simulink model "grid_forming_dq"  (R2026b)
settings: Solver=ode23tb  StopTime=param.sim.simlength  FixedStep=tc  MaxStep=param.glb_time.tc
values from neighbouring files (symbols this model uses):
  param = struct()    [init_model.m]
undefined symbols (not defined in the file or in its folder): magnitude
libraries: fl_lib x163, nesl_utility x93, igbt_simple_2th_lib x6, single_phase_transformer_lib x3, threephase_inductor_lib x2, dclink_for_two_levels x1, three_phase_pwm_modulator x1, lithium_ion_battery x1, three_phase_rl_load x1
(part 3 of 6)

== system grid_forming_dq/afe_dq_mod1/AFE_control/afe_control/current_ctrl/current_transformation ==
  is_a_pu : Inport
  is_b_pu : Inport  Port=2
  is_c_pu : Inport  Port=3
  alphabeta2xieta : MATLAB Function  TreatAsAtomicUnit=on
  uvw2alphabeta : MATLAB Function  TreatAsAtomicUnit=on
  tag scope: id_eta_pu=scoped, id_xi_pu=scoped
  wires:
  is_c_pu/1 -> uvw2alphabeta/3(w)
  alphabeta2xieta/2(eta) -> [id_eta_pu]  "ieta_pu"
  alphabeta2xieta/1(xi) -> [id_xi_pu]  "ixi_pu"
  is_b_pu/1 -> uvw2alphabeta/2(v)
  uvw2alphabeta/2(beta) -> alphabeta2xieta/2(beta)  "ibeta_pu"
  uvw2alphabeta/1(alpha) -> alphabeta2xieta/1(alpha)  "ialpha_pu"
  [phase_grid_pll] -> alphabeta2xieta/3(gamma)
  is_a_pu/1 -> uvw2alphabeta/1(u)

== system grid_forming_dq/afe_dq_mod1/AFE_control/afe_control/current_ctrl/dq_vector_pi ==
  id : Inport
  id_ref : Inport  Port=2
  iq : Inport  Port=3
  iq_ref : Inport  Port=4
  Sum1 : Sum  Inputs=|-+
  Sum2 : Sum  Inputs=|-+
  bounder1 : Subsystem
  bounder2 : Subsystem
  id/id_ref : Scope  NumInputPorts=2
      settings: ActiveDisplayYMinimum=-0.59440941888164511  ActiveDisplayYMaximum=1.5837925471243963  DataLoggingVariableName=ScopeData4
  iq/iq_ref : Scope  NumInputPorts=2
      settings: ActiveDisplayYMinimum=-1.3392283585411369  ActiveDisplayYMaximum=1.0516657066165265  DataLoggingVariableName=ScopeData5
  pi_d : Subsystem
  pi_q : Subsystem
  switch : Subsystem
  vector lenght : Subsystem
  md_sat : Outport
  mq_sat : Outport  Port=2
  wires:
  bounder2/2(clip) -> switch/2(clip 2)
  vector lenght/2(m) -> bounder1/3(m), bounder2/1(m)
  Sum2/1 -> pi_q/1(iq_tilde)
  pi_d/1(ud_ctrl_out) -> vector lenght/1(md), bounder1/1(md)
  pi_q/1(uq_ctrl_out) -> bounder2/3(mq), vector lenght/2(mq)
  vector lenght/1(m_1) -> bounder1/2(m_1), bounder2/2(m_1)
  switch/1(clip) -> pi_d/2(clip), pi_q/2(clip)
  iq/1 -> Sum2/1, iq/iq_ref/1  "iq"
  Sum1/1 -> pi_d/1(id_tilde)
  bounder1/2(clip) -> switch/1(clip 1)
  bounder1/1(md_sat) -> md_sat/1
  bounder2/1(mq_sat) -> mq_sat/1
  id_ref/1 -> id/id_ref/2, Sum1/2  "id_ref"
  iq_ref/1 -> iq/iq_ref/2, Sum2/2  "iq_ref"
  id/1 -> id/id_ref/1, Sum1/1  "id"

== system grid_forming_dq/afe_dq_mod1/AFE_control/afe_control/current_ctrl/zero_current_ctrl ==
  ualpha_ctrl_afe : Inport
  ubeta_ctrl_afe : Inport  Port=2
  Bus Creator1 : BusCreator  Inputs=3
  Constant : Constant  Value=0
  uabg_ctrl_out : Outport
  wires:
  Bus Creator1/1 -> uabg_ctrl_out/1
  ualpha_ctrl_afe/1 -> Bus Creator1/1  "ualpha_ctrl_afe"
  ubeta_ctrl_afe/1 -> Bus Creator1/2  "ubeta_ctrl_afe"
  Constant/1 -> Bus Creator1/3  "ugamma_ctrl_afe"

== system grid_forming_dq/afe_dq_mod1/AFE_control/afe_control/data_to_worspace_module_1/dq_pll ==
  Bus Creator1 : BusCreator  Inputs=8
  dqPLLs : Outport
  wires:
  [phase_grid_fht_simulink_pll] -> Bus Creator1/5  "phase_grid_fht_simulink_pll"
  [omega_grid_fht_simulink_pll] -> Bus Creator1/6  "omega_grid_fht_simulink_pll"
  [omega_grid_fhtsr_dqpll] -> Bus Creator1/8  "omega_grid_fhtsr_dqpll"
  [phase_grid_fhtsr_dqpll] -> Bus Creator1/7  "phase_grid_fhtsr_dqpll"
  [omega_grid_dqpll_ccaller] -> Bus Creator1/4  "omega_grid_dqpll_ccaller"
  [phase_grid_dqpll_ccaller] -> Bus Creator1/3  "phase_grid_dqpll_ccaller"
  [omega_grid_pu_dqpll] -> Bus Creator1/2  "omega_grid_pu_dqpll"
  [phase_grid_dqpll] -> Bus Creator1/1  "phase_grid_dqpll"
  Bus Creator1/1 -> dqPLLs/1

== system grid_forming_dq/afe_dq_mod1/AFE_control/afe_control/data_to_worspace_module_1/pwr_meter ==
  Bus Creator1 : BusCreator  Inputs=4
  m_pwr_meter : Outport
  wires:
  [u_grid_pu_rms] -> Bus Creator1/2  "u_grid_pu_rms"
  Bus Creator1/1 -> m_pwr_meter/1
  [pwr_act_grid] -> Bus Creator1/3  "pwr_act_grid"
  [pwr_react_grid] -> Bus Creator1/4  "pwr_react_grid"
  [i_grid_pu_rms] -> Bus Creator1/1  "i_grid_pu_rms"

== system grid_forming_dq/afe_dq_mod1/AFE_control/afe_control/dq_neg_vector_pi/bounder1 ==
  md : Inport
  m_1 : Inport  Port=2
  m : Inport  Port=3
  Constant : Constant
  Constant1 : Constant  Value=0
  Divide : Product
  Gain : Gain  Gain=param.afe.ctrl.ixi_pos_ref_lim
  Switch : Switch  Threshold=param.afe.ctrl.ixi_pos_ref_lim  SaturateOnIntegerOverflow=off  InputSameDT=off
  Switch1 : Switch  Threshold=param.afe.ctrl.ixi_pos_ref_lim  SaturateOnIntegerOverflow=off  InputSameDT=off
  md_sat : Outport  VectorParamsAs1DForOutWhenUnconnected=off
  clip : Outport  Port=2  VectorParamsAs1DForOutWhenUnconnected=off
  wires:
  Gain/1 -> Switch1/1
  Switch1/1 -> md_sat/1
  Constant1/1 -> Switch/3
  Constant/1 -> Switch/1
  m/1 -> Switch1/2, Switch/2
  Switch/1 -> clip/1
  Divide/1 -> Gain/1
  m_1/1 -> Divide/1
  md/1 -> Divide/2, Switch1/3

== system grid_forming_dq/afe_dq_mod1/AFE_control/afe_control/dq_neg_vector_pi/bounder2 ==
  m : Inport
  m_1 : Inport  Port=2
  mq : Inport  Port=3
  Constant : Constant
  Constant1 : Constant  Value=0
  Divide : Product
  Gain : Gain  Gain=param.afe.ctrl.ixi_pos_ref_lim
  Switch : Switch  Threshold=param.afe.ctrl.ixi_pos_ref_lim  SaturateOnIntegerOverflow=off  InputSameDT=off
  Switch1 : Switch  Threshold=param.afe.ctrl.ixi_pos_ref_lim  SaturateOnIntegerOverflow=off  InputSameDT=off
  mq_sat : Outport  VectorParamsAs1DForOutWhenUnconnected=off
  clip : Outport  Port=2  VectorParamsAs1DForOutWhenUnconnected=off
  wires:
  Gain/1 -> Switch1/1
  mq/1 -> Switch1/3, Divide/2
  m_1/1 -> Divide/1
  Divide/1 -> Gain/1
  Switch1/1 -> mq_sat/1
  Switch/1 -> clip/1
  m/1 -> Switch/2, Switch1/2
  Constant/1 -> Switch/1
  Constant1/1 -> Switch/3

== system grid_forming_dq/afe_dq_mod1/AFE_control/afe_control/dq_neg_vector_pi/pi_d ==
  id_tilde : Inport
  clip : Inport  Port=2
  1/Ti : Gain  Gain=param.afe.ctrl.kp_ug_ctrl  SaturateOnIntegerOverflow=on  OutDataTypeStr=Inherit: Same as input  ParamDataTypeStr=Inherit: Same as input
  Constant : Constant  Value=0
  Sum2 : Sum  Inputs=+-  SaturateOnIntegerOverflow=on
  Sum4 : Sum  SaturateOnIntegerOverflow=on
  Sum5 : Sum  SaturateOnIntegerOverflow=on
  Switch1 : Switch  Threshold=0.5  SaturateOnIntegerOverflow=off  InputSameDT=off
  Switch2 : Switch  Threshold=0.5  SaturateOnIntegerOverflow=off  InputSameDT=off
  Unit Delay1 : UnitDelay  SampleTime=-1
  Unit Delay2 : UnitDelay  SampleTime=-1
  kp1 : Gain  Gain=param.ctrl.CTRPIFF_CLIP_RELEASE*param.glb_time.ts_inv  SaturateOnIntegerOverflow=on  OutDataTypeStr=Inherit: Same as input  ParamDataTypeStr=Inherit: Same as input
  kp2 : Gain  Gain=param.afe.ctrl.ki_ug_ctrl*param.glb_time.ts_inv  SaturateOnIntegerOverflow=on  OutDataTypeStr=Inherit: Same as input  ParamDataTypeStr=Inherit: Same as input
  ud_out : Outport  VectorParamsAs1DForOutWhenUnconnected=off
  wires:
  Unit Delay1/1 -> [clip]
  Constant/1 -> Switch2/1
  [clip] -> Switch1/2
  [clip] -> Switch2/2
  clip/1 -> Unit Delay1/1
  kp2/1 -> Switch2/3
  Switch2/1 -> Sum4/1
  1/Ti/1 -> Sum5/1
  Unit Delay2/1 -> Sum2/1, kp1/1, Sum4/2
  Sum2/1 -> Switch1/1
  kp1/1 -> Sum2/2
  Sum4/1 -> Switch1/3, Sum5/2
  Switch1/1 -> Unit Delay2/1
  Sum5/1 -> ud_out/1
  id_tilde/1 -> 1/Ti/1, kp2/1

== system grid_forming_dq/afe_dq_mod1/AFE_control/afe_control/dq_neg_vector_pi/pi_q ==
  iq_tilde : Inport
  clip : Inport  Port=2
  1/Ti : Gain  Gain=param.afe.ctrl.kp_ug_ctrl  SaturateOnIntegerOverflow=on  OutDataTypeStr=Inherit: Same as input  ParamDataTypeStr=Inherit: Same as input
  Constant : Constant  Value=0
  Sum2 : Sum  Inputs=+-  SaturateOnIntegerOverflow=on
  Sum4 : Sum  SaturateOnIntegerOverflow=on
  Sum5 : Sum  SaturateOnIntegerOverflow=on
  Switch1 : Switch  Threshold=0.5  SaturateOnIntegerOverflow=off  InputSameDT=off
  Switch2 : Switch  Threshold=0.5  SaturateOnIntegerOverflow=off  InputSameDT=off
  Unit Delay1 : UnitDelay  SampleTime=-1
  Unit Delay2 : UnitDelay  SampleTime=-1
  kp1 : Gain  Gain=param.ctrl.CTRPIFF_CLIP_RELEASE*param.glb_time.ts_inv  SaturateOnIntegerOverflow=on  OutDataTypeStr=Inherit: Same as input  ParamDataTypeStr=Inherit: Same as input
  kp2 : Gain  Gain=param.afe.ctrl.ki_ug_ctrl*param.glb_time.ts_inv  SaturateOnIntegerOverflow=on  OutDataTypeStr=Inherit: Same as input  ParamDataTypeStr=Inherit: Same as input
  Vqs_out : Outport  VectorParamsAs1DForOutWhenUnconnected=off
  wires:
  Sum5/1 -> Vqs_out/1
  Unit Delay1/1 -> [clip]
  iq_tilde/1 -> kp2/1, 1/Ti/1
  Switch1/1 -> Unit Delay2/1
  Sum4/1 -> Switch1/3, Sum5/2
  kp1/1 -> Sum2/2
  Sum2/1 -> Switch1/1
  Unit Delay2/1 -> Sum4/2, kp1/1, Sum2/1
  1/Ti/1 -> Sum5/1
  Switch2/1 -> Sum4/1
  kp2/1 -> Switch2/3
  clip/1 -> Unit Delay1/1
  [clip] -> Switch2/2
  [clip] -> Switch1/2
  Constant/1 -> Switch2/1

== system grid_forming_dq/afe_dq_mod1/AFE_control/afe_control/dq_neg_vector_pi/switch ==
  clip 1 : Inport
  clip 2 : Inport  Port=2
  Constant4 : Constant
  Constant5 : Constant  Value=0
  Sum1 : Sum  SaturateOnIntegerOverflow=on
  Switch : Switch  Threshold=0.5  SaturateOnIntegerOverflow=off  InputSameDT=off
  clip : Outport  VectorParamsAs1DForOutWhenUnconnected=off
  wires:
  clip 2/1 -> Sum1/2
  clip 1/1 -> Sum1/1
  Sum1/1 -> Switch/2
  Constant4/1 -> Switch/1
  Switch/1 -> clip/1
  Constant5/1 -> Switch/3

== system grid_forming_dq/afe_dq_mod1/AFE_control/afe_control/dq_neg_vector_pi/vector lenght ==
  md : Inport
  mq : Inport  Port=2
  Math Function : Math  Operator=magnitude^2  SignedPower=on
  Math Function1 : Math  Operator=magnitude^2  SignedPower=on
  Math Function2 : Math  Operator=reciprocal  SignedPower=on
  Sqrt : Sqrt
  Sum5 : Sum  SaturateOnIntegerOverflow=on
  m_1 : Outport  VectorParamsAs1DForOutWhenUnconnected=off
  m : Outport  Port=2  VectorParamsAs1DForOutWhenUnconnected=off
  wires:
  md/1 -> Math Function/1
  Math Function2/1 -> m_1/1
  Sum5/1 -> Sqrt/1
  Math Function/1 -> Sum5/1
  Math Function1/1 -> Sum5/2
  mq/1 -> Math Function1/1
  Sqrt/1 -> Math Function2/1, m/1

== system grid_forming_dq/afe_dq_mod1/AFE_control/afe_control/dq_pos_vector_pi/bounder1 ==
  md : Inport
  m_1 : Inport  Port=2
  m : Inport  Port=3
  Constant : Constant
  Constant1 : Constant  Value=0
  Divide : Product
  Gain : Gain  Gain=param.afe.ctrl.ixi_pos_ref_lim
  Switch : Switch  Threshold=param.afe.ctrl.ixi_pos_ref_lim  SaturateOnIntegerOverflow=off  InputSameDT=off
  Switch1 : Switch  Threshold=param.afe.ctrl.ixi_pos_ref_lim  SaturateOnIntegerOverflow=off  InputSameDT=off
  md_sat : Outport  VectorParamsAs1DForOutWhenUnconnected=off
  clip : Outport  Port=2  VectorParamsAs1DForOutWhenUnconnected=off
  wires:
  md/1 -> Switch1/3, Divide/2
  m_1/1 -> Divide/1
  Divide/1 -> Gain/1
  Switch/1 -> clip/1
  m/1 -> Switch/2, Switch1/2
  Constant/1 -> Switch/1
  Constant1/1 -> Switch/3
  Switch1/1 -> md_sat/1
  Gain/1 -> Switch1/1

== system grid_forming_dq/afe_dq_mod1/AFE_control/afe_control/dq_pos_vector_pi/bounder2 ==
  m : Inport
  m_1 : Inport  Port=2
  mq : Inport  Port=3
  Constant : Constant
  Constant1 : Constant  Value=0
  Divide : Product
  Gain : Gain  Gain=param.afe.ctrl.ixi_pos_ref_lim
  Switch : Switch  Threshold=param.afe.ctrl.ixi_pos_ref_lim  SaturateOnIntegerOverflow=off  InputSameDT=off
  Switch1 : Switch  Threshold=param.afe.ctrl.ixi_pos_ref_lim  SaturateOnIntegerOverflow=off  InputSameDT=off
  mq_sat : Outport  VectorParamsAs1DForOutWhenUnconnected=off
  clip : Outport  Port=2  VectorParamsAs1DForOutWhenUnconnected=off
  wires:
  Constant1/1 -> Switch/3
  Constant/1 -> Switch/1
  m/1 -> Switch1/2, Switch/2
  Switch/1 -> clip/1
  Switch1/1 -> mq_sat/1
  Divide/1 -> Gain/1
  m_1/1 -> Divide/1
  mq/1 -> Divide/2, Switch1/3
  Gain/1 -> Switch1/1

== system grid_forming_dq/afe_dq_mod1/AFE_control/afe_control/dq_pos_vector_pi/pi_d ==
  id_tilde : Inport
  clip : Inport  Port=2
  1/Ti : Gain  Gain=param.afe.ctrl.kp_ug_ctrl  SaturateOnIntegerOverflow=on  OutDataTypeStr=Inherit: Same as input  ParamDataTypeStr=Inherit: Same as input
  Constant : Constant  Value=0
  Sum2 : Sum  Inputs=+-  SaturateOnIntegerOverflow=on
  Sum4 : Sum  SaturateOnIntegerOverflow=on
  Sum5 : Sum  SaturateOnIntegerOverflow=on
  Switch1 : Switch  Threshold=0.5  SaturateOnIntegerOverflow=off  InputSameDT=off
  Switch2 : Switch  Threshold=0.5  SaturateOnIntegerOverflow=off  InputSameDT=off
  Unit Delay1 : UnitDelay  SampleTime=-1
  Unit Delay2 : UnitDelay  SampleTime=-1
  kp1 : Gain  Gain=param.ctrl.CTRPIFF_CLIP_RELEASE*param.glb_time.ts_inv  SaturateOnIntegerOverflow=on  OutDataTypeStr=Inherit: Same as input  ParamDataTypeStr=Inherit: Same as input
  kp2 : Gain  Gain=param.afe.ctrl.ki_ug_ctrl*param.glb_time.ts_inv  SaturateOnIntegerOverflow=on  OutDataTypeStr=Inherit: Same as input  ParamDataTypeStr=Inherit: Same as input
  ud_out : Outport  VectorParamsAs1DForOutWhenUnconnected=off
  wires:
  id_tilde/1 -> kp2/1, 1/Ti/1
  Sum5/1 -> ud_out/1
  Switch1/1 -> Unit Delay2/1
  Sum4/1 -> Sum5/2, Switch1/3
  kp1/1 -> Sum2/2
  Sum2/1 -> Switch1/1
  Unit Delay2/1 -> Sum4/2, kp1/1, Sum2/1
  1/Ti/1 -> Sum5/1
  Switch2/1 -> Sum4/1
  kp2/1 -> Switch2/3
  clip/1 -> Unit Delay1/1
  [clip] -> Switch2/2
  [clip] -> Switch1/2
  Constant/1 -> Switch2/1
  Unit Delay1/1 -> [clip]

== system grid_forming_dq/afe_dq_mod1/AFE_control/afe_control/dq_pos_vector_pi/pi_q ==
  iq_tilde : Inport
  clip : Inport  Port=2
  1/Ti : Gain  Gain=param.afe.ctrl.kp_ug_ctrl  SaturateOnIntegerOverflow=on  OutDataTypeStr=Inherit: Same as input  ParamDataTypeStr=Inherit: Same as input
  Constant : Constant  Value=0
  Sum2 : Sum  Inputs=+-  SaturateOnIntegerOverflow=on
  Sum4 : Sum  SaturateOnIntegerOverflow=on
  Sum5 : Sum  SaturateOnIntegerOverflow=on
  Switch1 : Switch  Threshold=0.5  SaturateOnIntegerOverflow=off  InputSameDT=off
  Switch2 : Switch  Threshold=0.5  SaturateOnIntegerOverflow=off  InputSameDT=off
  Unit Delay1 : UnitDelay  SampleTime=-1
  Unit Delay2 : UnitDelay  SampleTime=-1
  kp1 : Gain  Gain=param.ctrl.CTRPIFF_CLIP_RELEASE*param.glb_time.ts_inv  SaturateOnIntegerOverflow=on  OutDataTypeStr=Inherit: Same as input  ParamDataTypeStr=Inherit: Same as input
  kp2 : Gain  Gain=param.afe.ctrl.ki_ug_ctrl*param.glb_time.ts_inv  SaturateOnIntegerOverflow=on  OutDataTypeStr=Inherit: Same as input  ParamDataTypeStr=Inherit: Same as input
  Vqs_out : Outport  VectorParamsAs1DForOutWhenUnconnected=off
  wires:
  Constant/1 -> Switch2/1
  [clip] -> Switch1/2
  [clip] -> Switch2/2
  clip/1 -> Unit Delay1/1
  kp2/1 -> Switch2/3
  Switch2/1 -> Sum4/1
  1/Ti/1 -> Sum5/1
  Unit Delay2/1 -> Sum2/1, kp1/1, Sum4/2
  Sum2/1 -> Switch1/1
  kp1/1 -> Sum2/2
  Sum4/1 -> Sum5/2, Switch1/3
  Switch1/1 -> Unit Delay2/1
  iq_tilde/1 -> 1/Ti/1, kp2/1
  Unit Delay1/1 -> [clip]
  Sum5/1 -> Vqs_out/1

== system grid_forming_dq/afe_dq_mod1/AFE_control/afe_control/dq_pos_vector_pi/switch ==
  clip 1 : Inport
  clip 2 : Inport  Port=2
  Constant4 : Constant
  Constant5 : Constant  Value=0
  Sum1 : Sum  SaturateOnIntegerOverflow=on
  Switch : Switch  Threshold=0.5  SaturateOnIntegerOverflow=off  InputSameDT=off
  clip : Outport  VectorParamsAs1DForOutWhenUnconnected=off
  wires:
  Constant5/1 -> Switch/3
  Switch/1 -> clip/1
  Constant4/1 -> Switch/1
  Sum1/1 -> Switch/2
  clip 1/1 -> Sum1/1
  clip 2/1 -> Sum1/2

== system grid_forming_dq/afe_dq_mod1/AFE_control/afe_control/dq_pos_vector_pi/vector lenght ==
  md : Inport
  mq : Inport  Port=2
  Math Function : Math  Operator=magnitude^2  SignedPower=on
  Math Function1 : Math  Operator=magnitude^2  SignedPower=on
  Math Function2 : Math  Operator=reciprocal  SignedPower=on
  Sqrt : Sqrt
  Sum5 : Sum  SaturateOnIntegerOverflow=on
  m_1 : Outport  VectorParamsAs1DForOutWhenUnconnected=off
  m : Outport  Port=2  VectorParamsAs1DForOutWhenUnconnected=off
  wires:
  Sqrt/1 -> m/1, Math Function2/1
  mq/1 -> Math Function1/1
  Math Function1/1 -> Sum5/2
  Math Function/1 -> Sum5/1
  Sum5/1 -> Sqrt/1
  Math Function2/1 -> m_1/1
  md/1 -> Math Function/1

== system grid_forming_dq/afe_dq_mod1/AFE_control/afe_control/grid_voltage_phase_lock_loops/FHT-PLL ==
  ug_abc_pu : Inport
  pll_stageA : Subsystem
  wires:
  ug_abc_pu/1 -> pll_stageA/2(ug_abc_pu)
  [phase_grid_pll] -> pll_stageA/1(gamma_grid)

== system grid_forming_dq/afe_dq_mod1/AFE_control/afe_control/grid_voltage_phase_lock_loops/phase-generator ==
  Constant : Constant  Value=param.grid.fgrid
  Constant1 : Constant  Value=0
  Constant2 : Constant  Value=param.glb_time.ts_afe
  Constant3 : Constant  Value=0
  MATLAB Function : MATLAB Function  TreatAsAtomicUnit=on
  normalization : Gain  Gain=1/param.grid.fgrid/2/pi
  tag scope: omega_grid_pll_pu=scoped, phase_grid_pll=scoped
  wires:
  Constant/1 -> MATLAB Function/1(f)
  Constant3/1 -> MATLAB Function/4(theta0)
  MATLAB Function/1(theta) -> [phase_grid_pll]
  normalization/1 -> [omega_grid_pll_pu]
  Constant1/1 -> MATLAB Function/2(rst)
  Constant2/1 -> MATLAB Function/3(Ts)
  MATLAB Function/2(omega) -> normalization/1

== system grid_forming_dq/afe_dq_mod1/afe/three_phase_inverter_with_igbt_simple_2th/three_phase_inverter_with_igbt_simple_2th/igbt_simple_1 ==
  note: P_sw
  Capacitor : fl_lib/Electrical/Electrical Elements/Capacitor  c=Csnubber_m F  r=Rsnubber_m Ohm  g=0 1/Ohm  i_specify=off  i_priority=None  i=0 A  i_nominal_specify=off  i_nominal_value=1  i_nominal_unit=A  v_specify=off  v_priority=None  v=0 V  v_nominal_specify=off  v_nominal_value=1  v_nominal_unit=V  vc_specify=off  vc_priority=High  vc=0 V  vc_nominal_specify=off  vc_nominal_value=1  vc_nominal_unit=V
  IGBT_simple : Subsystem
      settings: PortSchema="{\"entries\":[{\"content\":{\"sides\":[{\"content\":{\"connectorIds\":[\"LConn1\"]},\"type\":\"ConnectorPlacement.EquallySpacedRectSide\",\"uuid\":\"c3d88d60-081d-4221-ab18-079856838dba\"},{\"content\":{\"side\":\"RIGHT\"},\"type\":\"ConnectorPlacement.EquallySpacedRectSide\",\"uuid\":\"76e7d76c-8b60-4107-8aac-a7654bd886e1\"},{\"content\":{\"connectorIds\":[\"LConn2\"],\"side\":\"TOP\"},\"type\":\"ConnectorPlacement.EquallySpacedRectSide\",\"uuid\":\"fbef57e1-7143-4076-ada8-0654b1d9ee0b\"},{\"content\":{\"connectorIds\":[\"RConn1\"],\"side\":\"BOTTOM\"},\"type\":\"ConnectorPlacement.EquallySpacedRectSide\",\"uuid\":\"f2fea5db-9515-452a-a480-7d54bae36c49\"}]},\"type\":\"ConnectorPlacement.EquallySpacedConnector\",\"uuid\":\"cddff0b8-236e-4840-ad87-03abcdd65fe7\"}],\"packageUris\":[\"http://schema.mathworks.com/mf0/Connector/R2020b\"],\"version\":\"1.0\"}"
  Voltage Sensor : fl_lib/Electrical/Electrical Sensors/Voltage Sensor
  uph : nesl_utility/PS-Simulink Converter  PhysicalDomain=network_engine_domain  SubClassName=ps_output  LeftPortType=input  RightPortType=output  PseudoPeriodic=off  Frequencies=[]  VectorFormat=1-D array  Unit=V  AffineConversion=off
  G : PMIOPort  Side=Left
  C : PMIOPort  Port=2  Side=Left
  E : PMIOPort  Port=3  Side=Right
  tag scope: igbt_voltage_Q1=scoped
  wires:
  uph/1 -> [igbt_voltage_Q1]  "uph"
  connections:
  G/RConn1 -- IGBT_simple/LConn1
  Voltage Sensor/RConn1 -- uph/LConn1
  Capacitor/LConn1 -- Voltage Sensor/LConn1 -- C/RConn1 -- IGBT_simple/LConn2
  Capacitor/RConn1 -- Voltage Sensor/RConn2 -- E/RConn1 -- IGBT_simple/RConn1

== system grid_forming_dq/afe_dq_mod1/afe/three_phase_inverter_with_igbt_simple_2th/three_phase_inverter_with_igbt_simple_2th/igbt_simple_2 ==
  note: P_sw
  Capacitor : fl_lib/Electrical/Electrical Elements/Capacitor  c=Csnubber_m F  r=Rsnubber_m Ohm  g=0 1/Ohm  i_specify=off  i_priority=None  i=0 A  i_nominal_specify=off  i_nominal_value=1  i_nominal_unit=A  v_specify=off  v_priority=None  v=0 V  v_nominal_specify=off  v_nominal_value=1  v_nominal_unit=V  vc_specify=off  vc_priority=High  vc=0 V  vc_nominal_specify=off  vc_nominal_value=1  vc_nominal_unit=V
  IGBT_simple : Subsystem
      settings: PortSchema="{\"entries\":[{\"content\":{\"sides\":[{\"content\":{\"connectorIds\":[\"LConn1\"]},\"type\":\"ConnectorPlacement.EquallySpacedRectSide\",\"uuid\":\"c3d88d60-081d-4221-ab18-079856838dba\"},{\"content\":{\"side\":\"RIGHT\"},\"type\":\"ConnectorPlacement.EquallySpacedRectSide\",\"uuid\":\"76e7d76c-8b60-4107-8aac-a7654bd886e1\"},{\"content\":{\"connectorIds\":[\"LConn2\"],\"side\":\"TOP\"},\"type\":\"ConnectorPlacement.EquallySpacedRectSide\",\"uuid\":\"fbef57e1-7143-4076-ada8-0654b1d9ee0b\"},{\"content\":{\"connectorIds\":[\"RConn1\"],\"side\":\"BOTTOM\"},\"type\":\"ConnectorPlacement.EquallySpacedRectSide\",\"uuid\":\"f2fea5db-9515-452a-a480-7d54bae36c49\"}]},\"type\":\"ConnectorPlacement.EquallySpacedConnector\",\"uuid\":\"cddff0b8-236e-4840-ad87-03abcdd65fe7\"}],\"packageUris\":[\"http://schema.mathworks.com/mf0/Connector/R2020b\"],\"version\":\"1.0\"}"
  Voltage Sensor : fl_lib/Electrical/Electrical Sensors/Voltage Sensor
  uph : nesl_utility/PS-Simulink Converter  PhysicalDomain=network_engine_domain  SubClassName=ps_output  LeftPortType=input  RightPortType=output  PseudoPeriodic=off  Frequencies=[]  VectorFormat=1-D array  Unit=V  AffineConversion=off
  G : PMIOPort  Side=Left
  C : PMIOPort  Port=2  Side=Left
  E : PMIOPort  Port=3  Side=Right
  tag scope: igbt_voltage_Q2=scoped
  wires:
  uph/1 -> [igbt_voltage_Q2]  "uph"
  connections:
  IGBT_simple/RConn1 -- E/RConn1 -- Capacitor/RConn1 -- Voltage Sensor/RConn2
  C/RConn1 -- IGBT_simple/LConn2 -- Capacitor/LConn1 -- Voltage Sensor/LConn1
  Voltage Sensor/RConn1 -- uph/LConn1
  G/RConn1 -- IGBT_simple/LConn1

== system grid_forming_dq/afe_dq_mod1/afe/three_phase_inverter_with_igbt_simple_2th/three_phase_inverter_with_igbt_simple_2th/igbt_simple_3 ==
  note: P_sw
  Capacitor : fl_lib/Electrical/Electrical Elements/Capacitor  c=Csnubber_m F  r=Rsnubber_m Ohm  g=0 1/Ohm  i_specify=off  i_priority=None  i=0 A  i_nominal_specify=off  i_nominal_value=1  i_nominal_unit=A  v_specify=off  v_priority=None  v=0 V  v_nominal_specify=off  v_nominal_value=1  v_nominal_unit=V  vc_specify=off  vc_priority=High  vc=0 V  vc_nominal_specify=off  vc_nominal_value=1  vc_nominal_unit=V
  IGBT_simple : Subsystem
      settings: PortSchema="{\"entries\":[{\"content\":{\"sides\":[{\"content\":{\"connectorIds\":[\"LConn1\"]},\"type\":\"ConnectorPlacement.EquallySpacedRectSide\",\"uuid\":\"c3d88d60-081d-4221-ab18-079856838dba\"},{\"content\":{\"side\":\"RIGHT\"},\"type\":\"ConnectorPlacement.EquallySpacedRectSide\",\"uuid\":\"76e7d76c-8b60-4107-8aac-a7654bd886e1\"},{\"content\":{\"connectorIds\":[\"LConn2\"],\"side\":\"TOP\"},\"type\":\"ConnectorPlacement.EquallySpacedRectSide\",\"uuid\":\"fbef57e1-7143-4076-ada8-0654b1d9ee0b\"},{\"content\":{\"connectorIds\":[\"RConn1\"],\"side\":\"BOTTOM\"},\"type\":\"ConnectorPlacement.EquallySpacedRectSide\",\"uuid\":\"f2fea5db-9515-452a-a480-7d54bae36c49\"}]},\"type\":\"ConnectorPlacement.EquallySpacedConnector\",\"uuid\":\"cddff0b8-236e-4840-ad87-03abcdd65fe7\"}],\"packageUris\":[\"http://schema.mathworks.com/mf0/Connector/R2020b\"],\"version\":\"1.0\"}"
  Voltage Sensor : fl_lib/Electrical/Electrical Sensors/Voltage Sensor
  uph : nesl_utility/PS-Simulink Converter  PhysicalDomain=network_engine_domain  SubClassName=ps_output  LeftPortType=input  RightPortType=output  PseudoPeriodic=off  Frequencies=[]  VectorFormat=1-D array  Unit=V  AffineConversion=off
  G : PMIOPort  Side=Left
  C : PMIOPort  Port=2  Side=Left
  E : PMIOPort  Port=3  Side=Right
  tag scope: igbt_voltage_Q3=scoped
  wires:
  uph/1 -> [igbt_voltage_Q3]  "uph"
  connections:
  G/RConn1 -- IGBT_simple/LConn1
  Voltage Sensor/RConn1 -- uph/LConn1
  Voltage Sensor/LConn1 -- Capacitor/LConn1 -- IGBT_simple/LConn2 -- C/RConn1
  Voltage Sensor/RConn2 -- Capacitor/RConn1 -- E/RConn1 -- IGBT_simple/RConn1

== system grid_forming_dq/afe_dq_mod1/afe/three_phase_inverter_with_igbt_simple_2th/three_phase_inverter_with_igbt_simple_2th/igbt_simple_4 ==
  note: P_sw
  Capacitor : fl_lib/Electrical/Electrical Elements/Capacitor  c=Csnubber_m F  r=Rsnubber_m Ohm  g=0 1/Ohm  i_specify=off  i_priority=None  i=0 A  i_nominal_specify=off  i_nominal_value=1  i_nominal_unit=A  v_specify=off  v_priority=None  v=0 V  v_nominal_specify=off  v_nominal_value=1  v_nominal_unit=V  vc_specify=off  vc_priority=High  vc=0 V  vc_nominal_specify=off  vc_nominal_value=1  vc_nominal_unit=V
  IGBT_simple : Subsystem
      settings: PortSchema="{\"entries\":[{\"content\":{\"sides\":[{\"content\":{\"connectorIds\":[\"LConn1\"]},\"type\":\"ConnectorPlacement.EquallySpacedRectSide\",\"uuid\":\"c3d88d60-081d-4221-ab18-079856838dba\"},{\"content\":{\"side\":\"RIGHT\"},\"type\":\"ConnectorPlacement.EquallySpacedRectSide\",\"uuid\":\"76e7d76c-8b60-4107-8aac-a7654bd886e1\"},{\"content\":{\"connectorIds\":[\"LConn2\"],\"side\":\"TOP\"},\"type\":\"ConnectorPlacement.EquallySpacedRectSide\",\"uuid\":\"fbef57e1-7143-4076-ada8-0654b1d9ee0b\"},{\"content\":{\"connectorIds\":[\"RConn1\"],\"side\":\"BOTTOM\"},\"type\":\"ConnectorPlacement.EquallySpacedRectSide\",\"uuid\":\"f2fea5db-9515-452a-a480-7d54bae36c49\"}]},\"type\":\"ConnectorPlacement.EquallySpacedConnector\",\"uuid\":\"cddff0b8-236e-4840-ad87-03abcdd65fe7\"}],\"packageUris\":[\"http://schema.mathworks.com/mf0/Connector/R2020b\"],\"version\":\"1.0\"}"
  Voltage Sensor : fl_lib/Electrical/Electrical Sensors/Voltage Sensor
  uph : nesl_utility/PS-Simulink Converter  PhysicalDomain=network_engine_domain  SubClassName=ps_output  LeftPortType=input  RightPortType=output  PseudoPeriodic=off  Frequencies=[]  VectorFormat=1-D array  Unit=V  AffineConversion=off
  G : PMIOPort  Side=Left
  C : PMIOPort  Port=2  Side=Left
  E : PMIOPort  Port=3  Side=Right
  tag scope: igbt_voltage_Q4=scoped
  wires:
  uph/1 -> [igbt_voltage_Q4]  "uph"
  connections:
  IGBT_simple/RConn1 -- E/RConn1 -- Capacitor/RConn1 -- Voltage Sensor/RConn2
  C/RConn1 -- IGBT_simple/LConn2 -- Capacitor/LConn1 -- Voltage Sensor/LConn1
  Voltage Sensor/RConn1 -- uph/LConn1
  G/RConn1 -- IGBT_simple/LConn1

== system grid_forming_dq/afe_dq_mod1/afe/three_phase_inverter_with_igbt_simple_2th/three_phase_inverter_with_igbt_simple_2th/igbt_simple_5 ==
  note: P_sw
  Capacitor : fl_lib/Electrical/Electrical Elements/Capacitor  c=Csnubber_m F  r=Rsnubber_m Ohm  g=0 1/Ohm  i_specify=off  i_priority=None  i=0 A  i_nominal_specify=off  i_nominal_value=1  i_nominal_unit=A  v_specify=off  v_priority=None  v=0 V  v_nominal_specify=off  v_nominal_value=1  v_nominal_unit=V  vc_specify=off  vc_priority=High  vc=0 V  vc_nominal_specify=off  vc_nominal_value=1  vc_nominal_unit=V
  IGBT_simple : Subsystem
      settings: PortSchema="{\"entries\":[{\"content\":{\"sides\":[{\"content\":{\"connectorIds\":[\"LConn1\"]},\"type\":\"ConnectorPlacement.EquallySpacedRectSide\",\"uuid\":\"c3d88d60-081d-4221-ab18-079856838dba\"},{\"content\":{\"side\":\"RIGHT\"},\"type\":\"ConnectorPlacement.EquallySpacedRectSide\",\"uuid\":\"76e7d76c-8b60-4107-8aac-a7654bd886e1\"},{\"content\":{\"connectorIds\":[\"LConn2\"],\"side\":\"TOP\"},\"type\":\"ConnectorPlacement.EquallySpacedRectSide\",\"uuid\":\"fbef57e1-7143-4076-ada8-0654b1d9ee0b\"},{\"content\":{\"connectorIds\":[\"RConn1\"],\"side\":\"BOTTOM\"},\"type\":\"ConnectorPlacement.EquallySpacedRectSide\",\"uuid\":\"f2fea5db-9515-452a-a480-7d54bae36c49\"}]},\"type\":\"ConnectorPlacement.EquallySpacedConnector\",\"uuid\":\"cddff0b8-236e-4840-ad87-03abcdd65fe7\"}],\"packageUris\":[\"http://schema.mathworks.com/mf0/Connector/R2020b\"],\"version\":\"1.0\"}"
  Voltage Sensor : fl_lib/Electrical/Electrical Sensors/Voltage Sensor
  uph : nesl_utility/PS-Simulink Converter  PhysicalDomain=network_engine_domain  SubClassName=ps_output  LeftPortType=input  RightPortType=output  PseudoPeriodic=off  Frequencies=[]  VectorFormat=1-D array  Unit=V  AffineConversion=off
  G : PMIOPort  Side=Left
  C : PMIOPort  Port=2  Side=Left
  E : PMIOPort  Port=3  Side=Right
  tag scope: igbt_voltage_Q5=scoped
  wires:
  uph/1 -> [igbt_voltage_Q5]  "uph"
  connections:
  G/RConn1 -- IGBT_simple/LConn1
  Voltage Sensor/RConn1 -- uph/LConn1
  Voltage Sensor/LConn1 -- Capacitor/LConn1 -- IGBT_simple/LConn2 -- C/RConn1
  Voltage Sensor/RConn2 -- Capacitor/RConn1 -- E/RConn1 -- IGBT_simple/RConn1

== system grid_forming_dq/afe_dq_mod1/afe/three_phase_inverter_with_igbt_simple_2th/three_phase_inverter_with_igbt_simple_2th/igbt_simple_6 ==
  note: P_sw
  Capacitor : fl_lib/Electrical/Electrical Elements/Capacitor  c=Csnubber_m F  r=Rsnubber_m Ohm  g=0 1/Ohm  i_specify=off  i_priority=None  i=0 A  i_nominal_specify=off  i_nominal_value=1  i_nominal_unit=A  v_specify=off  v_priority=None  v=0 V  v_nominal_specify=off  v_nominal_value=1  v_nominal_unit=V  vc_specify=off  vc_priority=High  vc=0 V  vc_nominal_specify=off  vc_nominal_value=1  vc_nominal_unit=V
  IGBT_simple : Subsystem
      settings: PortSchema="{\"entries\":[{\"content\":{\"sides\":[{\"content\":{\"connectorIds\":[\"LConn1\"]},\"type\":\"ConnectorPlacement.EquallySpacedRectSide\",\"uuid\":\"c3d88d60-081d-4221-ab18-079856838dba\"},{\"content\":{\"side\":\"RIGHT\"},\"type\":\"ConnectorPlacement.EquallySpacedRectSide\",\"uuid\":\"76e7d76c-8b60-4107-8aac-a7654bd886e1\"},{\"content\":{\"connectorIds\":[\"LConn2\"],\"side\":\"TOP\"},\"type\":\"ConnectorPlacement.EquallySpacedRectSide\",\"uuid\":\"fbef57e1-7143-4076-ada8-0654b1d9ee0b\"},{\"content\":{\"connectorIds\":[\"RConn1\"],\"side\":\"BOTTOM\"},\"type\":\"ConnectorPlacement.EquallySpacedRectSide\",\"uuid\":\"f2fea5db-9515-452a-a480-7d54bae36c49\"}]},\"type\":\"ConnectorPlacement.EquallySpacedConnector\",\"uuid\":\"cddff0b8-236e-4840-ad87-03abcdd65fe7\"}],\"packageUris\":[\"http://schema.mathworks.com/mf0/Connector/R2020b\"],\"version\":\"1.0\"}"
  Voltage Sensor : fl_lib/Electrical/Electrical Sensors/Voltage Sensor
  uph : nesl_utility/PS-Simulink Converter  PhysicalDomain=network_engine_domain  SubClassName=ps_output  LeftPortType=input  RightPortType=output  PseudoPeriodic=off  Frequencies=[]  VectorFormat=1-D array  Unit=V  AffineConversion=off
  G : PMIOPort  Side=Left
  C : PMIOPort  Port=2  Side=Left
  E : PMIOPort  Port=3  Side=Right
  tag scope: igbt_voltage_Q6=scoped
  wires:
  uph/1 -> [igbt_voltage_Q6]  "uph"
  connections:
  IGBT_simple/RConn1 -- E/RConn1 -- Capacitor/RConn1 -- Voltage Sensor/RConn2
  C/RConn1 -- IGBT_simple/LConn2 -- Capacitor/LConn1 -- Voltage Sensor/LConn1
  Voltage Sensor/RConn1 -- uph/LConn1
  G/RConn1 -- IGBT_simple/LConn1

== system grid_forming_dq/afe_dq_mod1/afe/three_phase_inverter_with_igbt_simple_2th/three_phase_inverter_with_igbt_simple_2th/module_1 ==
  Bus Creator : BusCreator  Inputs=18
  m : Outport
  wires:
  [diode_HA_temp_Q1] -> Bus Creator/8  "diode_HA_temp_Q1"
  [igbt_voltage_Q2] -> Bus Creator/10  "igbt_voltage_Q2"
  [igbt_voltage_Q1] -> Bus Creator/2  "igbt_voltage_Q1"
  [igbt_ploss_Q2] -> Bus Creator/9  "igbt_ploss_Q2"
  [igbt_current_Q2] -> Bus Creator/11  "igbt_current_Q2"
  [diode_ploss_Q1] -> Bus Creator/6  "diode_ploss_Q1"
  [diode_JH_temp_Q1] -> Bus Creator/7  "diode_JH_temp_Q1"
  [igbt_HA_temp_Q1] -> Bus Creator/5  "igbt_HA_temp_Q1"
  [igbt_ploss_Q1] -> Bus Creator/1  "igbt_ploss_Q1"
  [diode_JH_temp_Q2] -> Bus Creator/15  "diode_JH_temp_Q2"
  [diode_HA_temp_Q2] -> Bus Creator/16  "diode_HA_temp_Q2"
  [diode_ploss_Q2] -> Bus Creator/14  "diode_ploss_Q2"
  [igbt_HA_temp_Q2] -> Bus Creator/13  "igbt_HA_temp_Q2"
  [igbt_JH_temp_Q2] -> Bus Creator/12  "igbt_JH_temp_Q2"
  [igbt_JH_temp_Q1] -> Bus Creator/4  "igbt_JH_temp_Q1"
  [igbt_current_Q1] -> Bus Creator/3  "igbt_current_Q1"
  Bus Creator/1 -> m/1  "module_1"
  [diode_current_Q1] -> Bus Creator/17  "diode_current_Q1"
  [diode_current_Q2] -> Bus Creator/18  "diode_current_Q2"

== system grid_forming_dq/afe_dq_mod1/afe/three_phase_inverter_with_igbt_simple_2th/three_phase_inverter_with_igbt_simple_2th/module_2 ==
  Bus Creator1 : BusCreator  Inputs=18
  m : Outport
  wires:
  [diode_HA_temp_Q4] -> Bus Creator1/16  "diode_HA_temp_Q4"
  [igbt_HA_temp_Q3] -> Bus Creator1/5  "igbt_HA_temp_Q3"
  [igbt_JH_temp_Q3] -> Bus Creator1/4  "igbt_JH_temp_Q3"
  [diode_ploss_Q3] -> Bus Creator1/6  "diode_ploss_Q3"
  [diode_JH_temp_Q4] -> Bus Creator1/15  "diode_JH_temp_Q4"
  [igbt_ploss_Q3] -> Bus Creator1/1  "igbt_ploss_Q3"
  [igbt_JH_temp_Q4] -> Bus Creator1/12  "igbt_JH_temp_Q4"
  [igbt_voltage_Q3] -> Bus Creator1/2  "igbt_voltage_Q3"
  [igbt_current_Q4] -> Bus Creator1/11  "igbt_current_Q4"
  [diode_HA_temp_Q3] -> Bus Creator1/8  "diode_HA_temp_Q3"
  [igbt_voltage_Q4] -> Bus Creator1/10  "igbt_voltage_Q4"
  [igbt_ploss_Q4] -> Bus Creator1/9  "igbt_ploss_Q4"
  [igbt_HA_temp_Q4] -> Bus Creator1/13  "igbt_HA_temp_Q4"
  [diode_JH_temp_Q3] -> Bus Creator1/7  "diode_JH_temp_Q3"
  [diode_ploss_Q4] -> Bus Creator1/14  "diode_ploss_Q4"
  [igbt_current_Q3] -> Bus Creator1/3  "igbt_current_Q3"
  Bus Creator1/1 -> m/1  "module_2"
  [diode_current_Q4] -> Bus Creator1/18  "diode_current_Q4"
  [diode_current_Q3] -> Bus Creator1/17  "diode_current_Q3"

== system grid_forming_dq/afe_dq_mod1/afe/three_phase_inverter_with_igbt_simple_2th/three_phase_inverter_with_igbt_simple_2th/module_3 ==
  Bus Creator1 : BusCreator  Inputs=18
  m : Outport
  wires:
  [diode_ploss_Q6] -> Bus Creator1/14  "diode_ploss_Q6"
  [igbt_HA_temp_Q5] -> Bus Creator1/5  "igbt_HA_temp_Q5"
  [igbt_voltage_Q6] -> Bus Creator1/10  "igbt_voltage_Q6"
  [igbt_voltage_Q5] -> Bus Creator1/2  "igbt_voltage_Q5"
  [igbt_JH_temp_Q6] -> Bus Creator1/12  "igbt_JH_temp_Q6"
  [igbt_current_Q6] -> Bus Creator1/11  "igbt_current_Q6"
  [diode_JH_temp_Q6] -> Bus Creator1/15  "diode_JH_temp_Q6"
  [diode_HA_temp_Q5] -> Bus Creator1/8  "diode_HA_temp_Q5"
  [igbt_ploss_Q5] -> Bus Creator1/1  "igbt_ploss_Q5"
  [igbt_ploss_Q6] -> Bus Creator1/9  "igbt_ploss_Q6"
  [igbt_current_Q5] -> Bus Creator1/3  "igbt_current_Q5"
  [diode_JH_temp_Q5] -> Bus Creator1/7  "diode_JH_temp_Q5"
  [igbt_JH_temp_Q5] -> Bus Creator1/4  "igbt_JH_temp_Q5"
  [diode_HA_temp_Q6] -> Bus Creator1/16  "diode_HA_temp_Q6"
  [igbt_HA_temp_Q6] -> Bus Creator1/13  "igbt_HA_temp_Q6"
  [diode_ploss_Q5] -> Bus Creator1/6  "diode_ploss_Q5"
  Bus Creator1/1 -> m/1  "module_3"
  [diode_current_Q6] -> Bus Creator1/18  "diode_current_Q6"
  [diode_current_Q5] -> Bus Creator1/17  "diode_current_Q5"

== system grid_forming_dq/afe_dq_mod1/AFE_control/afe_control/acquisitions/ig afe quantizzation and one step delay/ig afe quantizzation and one step delay ==
  ig_u_pu : Inport
  ig_v_pu : Inport  Port=2
  ig_w_pu : Inport  Port=3
  Gain4 : Gain  Gain=-1
  Gain5 : Gain  Gain=-1
  Gain6 : Gain  Gain=-1
  Quantizer1 : Quantizer  QuantizationInterval=param.meas.adc_quantization
  Quantizer2 : Quantizer  QuantizationInterval=param.meas.adc_quantization
  Quantizer4 : Quantizer  QuantizationInterval=param.meas.adc_quantization
  Unit Delay : UnitDelay  SampleTime=-1
  Unit Delay1 : UnitDelay  SampleTime=-1
  Unit Delay2 : UnitDelay  SampleTime=-1
  Zero-Order Hold : ZeroOrderHold  SampleTime=-1
  Zero-Order Hold1 : ZeroOrderHold  SampleTime=-1
  Zero-Order Hold2 : ZeroOrderHold  SampleTime=-1
  igd_u_pu : Outport
  igd_v_pu : Outport  Port=2
  igd_w_pu : Outport  Port=3
  wires:
  Quantizer1/1 -> Unit Delay1/1
  Quantizer4/1 -> Unit Delay/1
  Quantizer2/1 -> Unit Delay2/1
  ig_u_pu/1 -> Zero-Order Hold/1
  ig_v_pu/1 -> Zero-Order Hold1/1
  ig_w_pu/1 -> Zero-Order Hold2/1
  Unit Delay/1 -> Gain4/1
  Unit Delay1/1 -> Gain5/1
  Unit Delay2/1 -> Gain6/1
  Gain4/1 -> igd_u_pu/1
  Gain5/1 -> igd_v_pu/1
  Gain6/1 -> igd_w_pu/1
  Zero-Order Hold/1 -> Quantizer4/1
  Zero-Order Hold1/1 -> Quantizer1/1
  Zero-Order Hold2/1 -> Quantizer2/1

== system grid_forming_dq/afe_dq_mod1/AFE_control/afe_control/acquisitions/is afe quantizzation and one step delay/is afe quantizzation and one step delay ==
  is_u_pu : Inport
  is_v_pu : Inport  Port=2
  is_w_pu : Inport  Port=3
  Quantizer : Quantizer  QuantizationInterval=param.meas.adc_quantization
  Quantizer1 : Quantizer  QuantizationInterval=param.meas.adc_quantization
  Quantizer2 : Quantizer  QuantizationInterval=param.meas.adc_quantization
  Unit Delay : UnitDelay  SampleTime=-1
  Unit Delay1 : UnitDelay  SampleTime=-1
  Unit Delay2 : UnitDelay  SampleTime=-1
  Zero-Order Hold : ZeroOrderHold  SampleTime=-1
  Zero-Order Hold1 : ZeroOrderHold  SampleTime=-1
  Zero-Order Hold2 : ZeroOrderHold  SampleTime=-1
  isd_u_pu : Outport
  isd_v_pu : Outport  Port=2
  isd_w_pu : Outport  Port=3
  wires:
  Unit Delay/1 -> isd_u_pu/1
  Unit Delay1/1 -> isd_v_pu/1
  Unit Delay2/1 -> isd_w_pu/1
  Quantizer/1 -> Unit Delay/1
  Quantizer1/1 -> Unit Delay1/1
  Quantizer2/1 -> Unit Delay2/1
  is_u_pu/1 -> Zero-Order Hold/1
  is_v_pu/1 -> Zero-Order Hold1/1
  is_w_pu/1 -> Zero-Order Hold2/1
  Zero-Order Hold/1 -> Quantizer/1
  Zero-Order Hold1/1 -> Quantizer1/1
  Zero-Order Hold2/1 -> Quantizer2/1

== system grid_forming_dq/afe_dq_mod1/AFE_control/afe_control/acquisitions/phase_compensation_1/alignment_eval_afe1 ==
  local_time : Inport
  master_time : Inport  Port=2
  Constant : Constant  Value=0
  Gain : Gain  Gain=-1
  Sum : Sum  Inputs=|+-
  pi : Subsystem  mask{kp=param.ctrl.kp_align, ki=param.ctrl.ki_align*param.glb_time.ts_afe, lim_up=param.ctrl.lim_up_align, lim_down=param.ctrl.lim_down_align}
      mask prompts: ki "ki*ts"
      mask Display:
      | disp('pi()');
      | port_label('input', 1, 'u_ref');
      | port_label('input', 2, 'u');
      | port_label('output', 1, 'y');
  dp : Outport
  wires:
  master_time/1 -> Sum/1
  Sum/1 -> Gain/1
  Constant/1 -> pi/1(u_ref)
  local_time/1 -> Sum/2
  Gain/1 -> pi/2(u)
  pi/1(y) -> dp/1

== system grid_forming_dq/afe_dq_mod1/AFE_control/afe_control/acquisitions/ug afe quantizzation and one step delay/ug afe quantizzation and one step delay ==
  ug_u_pu : Inport
  ug_v_pu : Inport  Port=2
  ug_w_pu : Inport  Port=3
  Quantizer1 : Quantizer  QuantizationInterval=param.meas.adc_quantization
  Quantizer2 : Quantizer  QuantizationInterval=param.meas.adc_quantization
  Quantizer4 : Quantizer  QuantizationInterval=param.meas.adc_quantization
  Unit Delay : UnitDelay  SampleTime=-1
  Unit Delay1 : UnitDelay  SampleTime=-1
  Unit Delay2 : UnitDelay  SampleTime=-1
  Zero-Order Hold : ZeroOrderHold  SampleTime=-1
  Zero-Order Hold1 : ZeroOrderHold  SampleTime=-1
  Zero-Order Hold2 : ZeroOrderHold  SampleTime=-1
  ugd_u_pu : Outport
  ugd_v_pu : Outport  Port=2
  ugd_w_pu : Outport  Port=3
  wires:
  Unit Delay/1 -> ugd_u_pu/1
  Unit Delay1/1 -> ugd_v_pu/1
  Unit Delay2/1 -> ugd_w_pu/1
  Quantizer4/1 -> Unit Delay/1
  Quantizer1/1 -> Unit Delay1/1
  Quantizer2/1 -> Unit Delay2/1
  ug_w_pu/1 -> Zero-Order Hold2/1
  ug_v_pu/1 -> Zero-Order Hold1/1
  ug_u_pu/1 -> Zero-Order Hold/1
  Zero-Order Hold/1 -> Quantizer4/1
  Zero-Order Hold1/1 -> Quantizer1/1
  Zero-Order Hold2/1 -> Quantizer2/1

== system grid_forming_dq/afe_dq_mod1/AFE_control/afe_control/current_ctrl/dq_vector_pi/bounder1 ==
  md : Inport
  m_1 : Inport  Port=2
  m : Inport  Port=3
  Constant : Constant
  Constant1 : Constant  Value=0
  Divide : Product
  Switch : Switch  Threshold=1  SaturateOnIntegerOverflow=off  InputSameDT=off
  Switch1 : Switch  Threshold=1  SaturateOnIntegerOverflow=off  InputSameDT=off
  md_sat : Outport  VectorParamsAs1DForOutWhenUnconnected=off
  clip : Outport  Port=2  VectorParamsAs1DForOutWhenUnconnected=off
  wires:
  md/1 -> Switch1/3, Divide/2
  m_1/1 -> Divide/1
  Divide/1 -> Switch1/1
  Switch1/1 -> md_sat/1
  Switch/1 -> clip/1
  m/1 -> Switch/2, Switch1/2
  Constant/1 -> Switch/1
  Constant1/1 -> Switch/3

== system grid_forming_dq/afe_dq_mod1/AFE_control/afe_control/current_ctrl/dq_vector_pi/bounder2 ==
  m : Inport
  m_1 : Inport  Port=2
  mq : Inport  Port=3
  Constant : Constant
  Constant1 : Constant  Value=0
  Divide : Product
  Switch : Switch  Threshold=1  SaturateOnIntegerOverflow=off  InputSameDT=off
  Switch1 : Switch  Threshold=1  SaturateOnIntegerOverflow=off  InputSameDT=off
  mq_sat : Outport  VectorParamsAs1DForOutWhenUnconnected=off
  clip : Outport  Port=2  VectorParamsAs1DForOutWhenUnconnected=off
  wires:
  Constant1/1 -> Switch/3
  Constant/1 -> Switch/1
  m/1 -> Switch1/2, Switch/2
  Switch/1 -> clip/1
  Switch1/1 -> mq_sat/1
  Divide/1 -> Switch1/1
  m_1/1 -> Divide/1
  mq/1 -> Divide/2, Switch1/3

== system grid_forming_dq/afe_dq_mod1/AFE_control/afe_control/current_ctrl/dq_vector_pi/pi_d ==
  id_tilde : Inport
  clip : Inport  Port=2
  1/Ti : Gain  Gain=param.afe.dq_vector_pi.kp_i  SaturateOnIntegerOverflow=on  OutDataTypeStr=Inherit: Same as input  ParamDataTypeStr=Inherit: Same as input
  Constant : Constant  Value=0
  Sum2 : Sum  Inputs=+-  SaturateOnIntegerOverflow=on
  Sum4 : Sum  SaturateOnIntegerOverflow=on
  Sum5 : Sum  Inputs=+++  SaturateOnIntegerOverflow=on
  Switch1 : Switch  Threshold=0.5  SaturateOnIntegerOverflow=off  InputSameDT=off
  Switch2 : Switch  Threshold=0.5  SaturateOnIntegerOverflow=off  InputSameDT=off
  Unit Delay1 : UnitDelay  SampleTime=-1
  Unit Delay2 : UnitDelay  SampleTime=-1
  kp1 : Gain  Gain=param.ctrl.CTRPIFF_CLIP_RELEASE*param.glb_time.ts_inv  SaturateOnIntegerOverflow=on  OutDataTypeStr=Inherit: Same as input  ParamDataTypeStr=Inherit: Same as input
  kp2 : Gain  Gain=param.afe.dq_vector_pi.ki_i*param.glb_time.ts_inv  SaturateOnIntegerOverflow=on  OutDataTypeStr=Inherit: Same as input  ParamDataTypeStr=Inherit: Same as input
  rpi_phase_d : Subsystem
  ud_ctrl_out : Outport  VectorParamsAs1DForOutWhenUnconnected=off
  wires:
  id_tilde/1 -> kp2/1, rpi_phase_d/1(id_tilde), 1/Ti/1
  Sum5/1 -> ud_ctrl_out/1
  Switch1/1 -> Unit Delay2/1
  Sum4/1 -> Sum5/2, Switch1/3
  kp1/1 -> Sum2/2
  Sum2/1 -> Switch1/1
  Unit Delay2/1 -> Sum4/2, kp1/1, Sum2/1
  1/Ti/1 -> Sum5/1
  Switch2/1 -> Sum4/1
  kp2/1 -> Switch2/3
  clip/1 -> Unit Delay1/1
  [clip] -> Switch2/2
  [clip] -> Switch1/2
  Constant/1 -> Switch2/1
  Unit Delay1/1 -> [clip]
  rpi_phase_d/1(Out1) -> Sum5/3

== system grid_forming_dq/afe_dq_mod1/AFE_control/afe_control/current_ctrl/dq_vector_pi/pi_q ==
  iq_tilde : Inport
  clip : Inport  Port=2
  1/Ti : Gain  Gain=param.afe.dq_vector_pi.kp_i  SaturateOnIntegerOverflow=on  OutDataTypeStr=Inherit: Same as input  ParamDataTypeStr=Inherit: Same as input
  Constant : Constant  Value=0
  Sum2 : Sum  Inputs=+-  SaturateOnIntegerOverflow=on
  Sum4 : Sum  SaturateOnIntegerOverflow=on
  Sum5 : Sum  Inputs=+++  SaturateOnIntegerOverflow=on
  Switch1 : Switch  Threshold=0.5  SaturateOnIntegerOverflow=off  InputSameDT=off
  Switch2 : Switch  Threshold=0.5  SaturateOnIntegerOverflow=off  InputSameDT=off
  Unit Delay1 : UnitDelay  SampleTime=-1
  Unit Delay2 : UnitDelay  SampleTime=-1
  kp1 : Gain  Gain=param.ctrl.CTRPIFF_CLIP_RELEASE*param.glb_time.ts_inv  SaturateOnIntegerOverflow=on  OutDataTypeStr=Inherit: Same as input  ParamDataTypeStr=Inherit: Same as input
  kp2 : Gain  Gain=param.afe.dq_vector_pi.ki_i*param.glb_time.ts_inv  SaturateOnIntegerOverflow=on  OutDataTypeStr=Inherit: Same as input  ParamDataTypeStr=Inherit: Same as input
  rpi_phase_q : Subsystem
  uq_ctrl_out : Outport  VectorParamsAs1DForOutWhenUnconnected=off
  wires:
  Constant/1 -> Switch2/1
  [clip] -> Switch1/2
  [clip] -> Switch2/2
  clip/1 -> Unit Delay1/1
  kp2/1 -> Switch2/3
  Switch2/1 -> Sum4/1
  1/Ti/1 -> Sum5/1
  Unit Delay2/1 -> Sum2/1, kp1/1, Sum4/2
  Sum2/1 -> Switch1/1
  kp1/1 -> Sum2/2
  Sum4/1 -> Sum5/2, Switch1/3
  Switch1/1 -> Unit Delay2/1
  Unit Delay1/1 -> [clip]
  Sum5/1 -> uq_ctrl_out/1
  iq_tilde/1 -> rpi_phase_q/1(id_tilde), 1/Ti/1, kp2/1
  rpi_phase_q/1(Out1) -> Sum5/3

== system grid_forming_dq/afe_dq_mod1/AFE_control/afe_control/current_ctrl/dq_vector_pi/switch ==
  clip 1 : Inport
  clip 2 : Inport  Port=2
  Constant4 : Constant
  Constant5 : Constant  Value=0
  Sum1 : Sum  SaturateOnIntegerOverflow=on
  Switch : Switch  Threshold=0.5  SaturateOnIntegerOverflow=off  InputSameDT=off
  clip : Outport  VectorParamsAs1DForOutWhenUnconnected=off
  wires:
  Constant5/1 -> Switch/3
  Switch/1 -> clip/1
  Constant4/1 -> Switch/1
  Sum1/1 -> Switch/2
  clip 1/1 -> Sum1/1
  clip 2/1 -> Sum1/2

== system grid_forming_dq/afe_dq_mod1/AFE_control/afe_control/current_ctrl/dq_vector_pi/vector lenght ==
  md : Inport
  mq : Inport  Port=2
  Math Function : Math  Operator=magnitude^2  SignedPower=on
  Math Function1 : Math  Operator=magnitude^2  SignedPower=on
  Math Function2 : Math  Operator=reciprocal  SignedPower=on
  Sqrt : Sqrt
  Sum5 : Sum  SaturateOnIntegerOverflow=on
  m_1 : Outport  VectorParamsAs1DForOutWhenUnconnected=off
  m : Outport  Port=2  VectorParamsAs1DForOutWhenUnconnected=off
  wires:
  Sqrt/1 -> m/1, Math Function2/1
  mq/1 -> Math Function1/1
  Math Function1/1 -> Sum5/2
  Math Function/1 -> Sum5/1
  Sum5/1 -> Sqrt/1
  Math Function2/1 -> m_1/1
  md/1 -> Math Function/1

== system grid_forming_dq/afe_dq_mod1/AFE_control/afe_control/grid_voltage_phase_lock_loops/FHT-PLL/pll_stageA ==
  gamma_grid : Inport
  ug_abc_pu : Inport  Port=2
  Demux : Demux  Outputs=3
  Math Function : Math  Operator=magnitude^2  SignedPower=on
  Math Function1 : Math  Operator=magnitude^2  SignedPower=on
  Scope : Scope  NumInputPorts=4
      settings: DataLoggingVariableName=ScopeData6
  Sqrt : Sqrt
  Sum : Sum  Inputs=|++
  filter_and_transformation : Subsystem
  sequences : Subsystem
  tag scope: u_grid_eta_n_pu=scoped, u_grid_eta_p_pu=scoped, u_grid_magnitude=scoped, u_grid_xi_n_pu=scoped, u_grid_xi_p_pu=scoped
  wires:
  gamma_grid/1 -> sequences/5(phase_angle)
  ug_abc_pu/1 -> Demux/1
  Demux/1 -> filter_and_transformation/1(ug_a)
  Demux/2 -> filter_and_transformation/2(ug_b)
  Demux/3 -> filter_and_transformation/3(ug_c)
  filter_and_transformation/1(ug_alpha_p) -> Math Function/1, sequences/1(u_grid_alpha_p), Scope/1  "ug_alpha_p"
  filter_and_transformation/2(ug_beta_p) -> Scope/2, Math Function1/1, sequences/2(u_grid_beta_p)  "ug_beta_p"
  Math Function/1 -> Sum/1
  Math Function1/1 -> Sum/2
  Sum/1 -> Sqrt/1
  sequences/1(u_grid_xi_p) -> [u_grid_xi_p_pu]
  sequences/2(u_grid_eta_p) -> [u_grid_eta_p_pu]
  Sqrt/1 -> [u_grid_magnitude]
  filter_and_transformation/3(ug_alpha_n) -> sequences/3(u_grid_alpha_n), Scope/3  "ug_alpha_n"
  filter_and_transformation/4(ug_beta_n) -> Scope/4, sequences/4(u_grid_beta_n)  "ug_beta_n"
  sequences/3(u_grid_xi_n) -> [u_grid_xi_n_pu]
  sequences/4(u_grid_eta_n) -> [u_grid_eta_n_pu]
